simulink model "gtm_design"  (R2021b)
settings: Solver=VariableStepAuto  StartTime=0.0  StopTime=30  MinStep=0.0049  RelTol=1e-3
StopFcn:
  | MWSout=grabmws(bdroot);
  | MWSout.lastrun=datestr(now);
values from neighbouring files (symbols this model uses):
  g = 32.17405    [SingleDOF.m]    (also in layer1atm.m; mainSimple.m = 32.174; simio.m = [dx(Index.EOM(1:6)); delta(:)-f; -delta(:)-f ])
  GuidanceMode = 1    [mainSimple.m]    (also in setup.m)
  knots2fps = 1/fps2knots    (= 1.687800745)    [main.m]    (also in mainSimple.m = 1.68781)
  s = tf('s')    [SingleDOF.m]    (also in main.m; mainSimple.m; newmain.m)
undefined symbols (not defined in the file or in its folder): Aero, aftfuel, aftfuel_pos, AILL, AILLC, AILR, AILRC, alpha_deg, altitude_ft, Ax_g, Ay_g, Az_g, b, beta_deg, bias, BRAKEC, Cbar, cg_pos0, cg_shift_gear, DamageCase, DamageModels, DamageOnsetTime, Earth, ELLIB, ELLIBC, ELLOB, ELLOBC, ELRIB, ELRIBC, ELROB, ELROBC, engl_ang, engl_pos, engr_ang, engr_pos, FLAPLC, FLAPLIB, FLAPLOB, FLAPRC, FLAPRIB, FLAPROB, FuelUsed_Init, fwdfuel, fwdfuel_pos, GEAR, GEARC, Inertia0, Inertia_shift_gear, Ixx_model, Iyy_model, Izz_model, KTAS, LandingGear, LengON, LinearizeModeOn, m, MORPHLC, MORPHRC, NAV_altitude_m, NAV_latitude_deg ... (+51)
libraries: simulink_extras x39, simulink_need_slupdate x30, LPVBlockLibrary x9, aerolibconvert2 x7, simulink x3, aerolibtransform2 x3, UserContent_lib x2, uavalgslib x2, robotcorelib x1, uavutilslib x1
(part 2 of 7)

== system gtm_design/GTM_T2/Landing Gear ==
  State : Inport
  Surfaces : Inport  Port=2
  ACParams : Inport  Port=3
  Bus Selector : BusSelector  OutputSignals=BRAKE,STEER,GEAR
  Bus Selector1 : BusSelector  OutputSignals=pb,qb,rb  OutputAsBus=on
  Bus Selector2 : BusSelector  OutputSignals=ub,vb,wb  OutputAsBus=on
  Bus Selector3 : BusSelector  OutputSignals=psi
  Bus Selector4 : BusSelector  OutputSignals=altitude
  Bus Selector5 : BusSelector  OutputSignals=phi,theta,psi  OutputAsBus=on
  Bus Selector6 : BusSelector  OutputSignals=CG  OutputAsBus=on
  Bus to Vector : BusToVector
  Bus to Vector1 : BusToVector
  Bus to Vector2 : BusToVector
  Gain : Gain  Gain=1/100
  LandingGear : Subsystem  mask{NoseWheelPos=LandingGear.NoseWheelPos, LeftMainPos=LandingGear.LeftMainPos, RightMainPos=LandingGear.RightMainPos, SpringConst=LandingGear.SpringConst, DampingConst=LandingGear.DampingConst, StrokeLength=LandingGear.StrokeLength, MountStiffness=LandingGear.MountStiff, MountDamping=LandingGear.MountDamping, RunwayAlt=runway_alt}
      mask prompts: NoseWheelPos "Nose Wheel Position [X,Y,Z]"; LeftMainPos "Left Main Position [X,Y,Z]"; RightMainPos "Right Main Position [X,Y,Z]"; SpringConst "Spring Constant [Nose,Left,Right]"; DampingConst "Damping Constant [Nose,Left,Right]"; StrokeLength "Stroke Length [Nose,Left,Right]"; MountStiffness "Mount Stiffness [Nose,Left,Right]"; MountDamping "Mount Damping [Nose,Left, Right]"; RunwayAlt "Runway Altitude"
      mask help:
      | Implements ground reaction force (if geardown is nonzero) for 3-wheel landing gear. Linear stiffness and damping are applied within stroke range, and (generally larger) mount stiffness and damping are applied beyond this range.
      |
      | Underlying gear.c function is from HL-20/LaRCsim, e.b.jackson@nasa.gov
  Mux : Mux  Inputs=2
  FM : Outport
  GearState : Outport  Port=2
  wires:
  Mux/1 -> FM/1
  Gain/1 -> LandingGear/7(Brake (0-1))
  LandingGear/3(Contact) -> GearState/1
  LandingGear/2(M_gear) -> Mux/2
  LandingGear/1(F_gear) -> Mux/1
  Bus Selector/3 -> LandingGear/9(geardown (0/1))  "<GEAR>"
  Bus Selector/2 -> LandingGear/8(Steer (deg))  "<STEER>"
  Bus Selector/1 -> Gain/1  "<BRAKE>"
  Bus Selector3/1 -> LandingGear/6(Heading (Rad))  "<psi>"
  Bus to Vector/1 -> LandingGear/4(pqr (Rad/sec))
  Bus Selector4/1 -> LandingGear/3(Altitude (ft))  "<altitude>"
  Bus to Vector2/1 -> LandingGear/2(EulerAngles (Rad))
  Bus Selector6/1 -> LandingGear/1(cg)
  Surfaces/1 -> Bus Selector/1
  State/1 -> Bus Selector1/1, Bus Selector2/1, Bus Selector3/1, Bus Selector4/1, Bus Selector5/1
  Bus Selector1/1 -> Bus to Vector/1
  Bus to Vector1/1 -> LandingGear/5(Vbody (ft/sec))
  Bus Selector2/1 -> Bus to Vector1/1
  Bus Selector5/1 -> Bus to Vector2/1
  ACParams/1 -> Bus Selector6/1

== system gtm_design/GTM_T2/Sensors ==
  EOM_State : Inport
  EOM_Xdot : Inport  Port=2
  AC_Params : Inport  Port=3
  AuxVars : Inport  Port=4
  SurfacePos : Inport  Port=5
  Engines : Inport  Port=6
  Air Data : Subsystem
  AuxVars1 : InportShadow  Port=4
  Bus Creator : BusCreator  Inputs=5
  Engine ECU 8 Hz : Subsystem  SystemSampleTime=round(1/Timestep/8)*Timestep
  MAG3 IMU : Subsystem
  MIDG II 50 Hz : Subsystem  SystemSampleTime=round(1/Timestep/50)*Timestep
  Scope{,1..4} (5 alike) : Scope
  Surface Pots : Subsystem
  Terminator : Terminator
  Terminator1 : Terminator
  Sensors : Outport
  wires:
  AC_Params/1 -> Terminator1/1
  EOM_Xdot/1 -> Terminator/1
  Bus Creator/1 -> Sensors/1
  Air Data/1(AirData) -> Scope/1, Bus Creator/1  "AirData"
  MIDG II 50 Hz/1(MIDG) -> Scope1/1, Bus Creator/2  "MIDG"
  Surface Pots/1(Pots) -> Scope3/1, Bus Creator/4  "SurfacePos"
  Engine ECU 8 Hz/1(ECU) -> Scope4/1, Bus Creator/5  "Engines"
  MAG3 IMU/1(MAG3) -> Scope2/1, Bus Creator/3  "MAG3"
  Engines/1 -> Engine ECU 8 Hz/1(Engines)
  SurfacePos/1 -> Surface Pots/1(SurfacePos)
  AuxVars/1 -> Air Data/2(AuxVars), MIDG II 50 Hz/1(AuxVars)
  EOM_State/1 -> MIDG II 50 Hz/2(EOM_State), Air Data/1(EOM_State), MAG3 IMU/2(EOM_State)
  AuxVars1/1 -> MAG3 IMU/1(AuxVars)

== system gtm_design/GTM_T2/TransportDelay ==
  note: Uplink Path
  note: Downlink Path
  Sensors : Inport
  UL : Inport  Port=2
  AntiAliasing : Subsystem
  Transport Delay on Bus : Subsystem
  Transport Delay on Bus1 : Subsystem
  cmds : Outport
  DL : Outport  Port=2
  wires:
  AntiAliasing/1(O) -> Transport Delay on Bus/1(In)
  Transport Delay on Bus/1(Out) -> DL/1
  UL/1 -> Transport Delay on Bus1/1(In)
  Sensors/1 -> AntiAliasing/1(I)
  Transport Delay on Bus1/1(Out) -> cmds/1

== system gtm_design/Guidance/Airspeed Step ==
  Action Port : ActionPort  ActionPortLabel=case [ 3 ]:
  Bus Creator : BusCreator  Inputs=5
  Constant1 : Constant  Value=-12.5
  Constant2 : Constant  Value=0
  Constant3 : Constant  Value=0
  Constant4 : Constant  Value=0
  Step1 : Step  Time=5  Before=85  After=90  SampleTime=0
  GuidanceCommand : Outport  InitialOutput=zeros(5,1)
  wires:
  Constant2/1 -> Bus Creator/2  "alt_c_ft"
  Constant4/1 -> Bus Creator/4  "phi_c_deg"
  Bus Creator/1 -> GuidanceCommand/1
  Constant3/1 -> Bus Creator/3  "bet_c_deg"
  Step1/1 -> Bus Creator/1  "tas_c_knot"
  Constant1/1 -> Bus Creator/5  "etas_c_percent"

== system gtm_design/Guidance/Elevation Step ==
  Action Port : ActionPort  ActionPortLabel=case [ 2 ]:
  Bus Creator : BusCreator  Inputs=5
  Constant : Constant  Value=85
  Constant1 : Constant  Value=-12.5
  Constant3 : Constant  Value=0
  Constant4 : Constant  Value=0
  Step : Step  Time=5  After=10  SampleTime=0
  GuidanceCommand : Outport  InitialOutput=zeros(5,1)
  wires:
  Constant/1 -> Bus Creator/1  "tas_c_knot"
  Constant1/1 -> Bus Creator/5  "etas_c_percent"
  Constant3/1 -> Bus Creator/3  "bet_c_deg"
  Constant4/1 -> Bus Creator/4  "phi_c_deg"
  Bus Creator/1 -> GuidanceCommand/1
  Step/1 -> Bus Creator/2  "alt_c_ft"

== system gtm_design/Guidance/Invalid, Error Out ==
  Action Port : ActionPort  ActionPortLabel=default:
  Constant1 : Constant  Value=zeros(5,1)
  Constant2 : Constant  Value=0
  InvalidMode : Assertion  AssertionFailFcn="warndlg('Invalid settings for TrimMode and LinearizeMode.  Run setup.m to reset.','Warning!')"
  Out : Outport  InitialOutput=zeros(5,1)
  wires:
  Constant1/1 -> Out/1
  Constant2/1 -> InvalidMode/1

== system gtm_design/Guidance/Label ==
  I : Inport  PortDimensions=[5 1]
  Bus Creator : BusCreator  Inputs=5
  Demux : Demux  Outputs=5
  O : Outport
  wires:
  Demux/4 -> Bus Creator/4  "phi_c_deg"
  Demux/2 -> Bus Creator/2  "alt_c_ft"
  Demux/5 -> Bus Creator/5  "etas_c_percent"
  Demux/3 -> Bus Creator/3  "bet_c_deg"
  Demux/1 -> Bus Creator/1  "tas_c_knot"
  Bus Creator/1 -> O/1
  I/1 -> Demux/1

== system gtm_design/Guidance/Level Flight ==
  Action Port : ActionPort  ActionPortLabel=case [ 1 ]:
  Bus Creator : BusCreator  Inputs=5
  Constant : Constant  Value=85
  Constant1 : Constant  Value=-12.5
  Constant2 : Constant  Value=0
  Constant3 : Constant  Value=0
  Constant4 : Constant  Value=0
  GuidanceCommand : Outport  InitialOutput=zeros(5,1)
  wires:
  Bus Creator/1 -> GuidanceCommand/1
  Constant3/1 -> Bus Creator/3  "bet_c_deg"
  Constant/1 -> Bus Creator/1  "tas_c_knot"
  Constant1/1 -> Bus Creator/5  "etas_c_percent"
  Constant4/1 -> Bus Creator/4  "phi_c_deg"
  Constant2/1 -> Bus Creator/2  "alt_c_ft"

== system gtm_design/Guidance/Orbit Following ==
  Feedback : Inport
  Action Port : ActionPort  ActionPortLabel=case [ 6 ]:
  Bus Creator : BusCreator  Inputs=5
  Bus Selector : BusSelector  OutputSignals=North,East,Height,HeadingAngle
  Constant : Constant  Value=80
  Constant1 : Constant  Value=-12.5
  Constant2 : Constant
  Constant3 : Constant  Value=0
  Constant4 : Constant  Value=1000
  Constant5 : Constant  Value=2000
  Gain2 : Gain  Gain=-1
  Gain5 : Gain  Gain=-1
  Heading Control : MATLAB Function  TreatAsAtomicUnit=on  mask(Fixed Wing Heading Controller){PHeadingAngle=3.9}
      mask prompts: PHeadingAngle "Heading Control Gain"
      mask help: P controller that regulates fixed wing UAV heading direction through controlling its roll angle. This controller requires that the plane is flying under coordinated flight condition.
  Length Conversion : aerolibconvert2/Length Conversion  IU=m  OU=ft
  Orbit Follower : uavalgslib/Orbit Follower  UAVType=fixed-wing  MinOrbitRadius=1  MinLookaheadDistance=0.1  ExternalReset=none  ShowCrossTrackErrorOutput=off  ShowNumTurnsOutput=off  SimulateUsing=Interpreted execution
      settings: SourceProductBaseCode=UV
  Radians to Degrees : simulink_extras/Transformations/Radians to Degrees
  Saturation1 : Saturate  UpperLimit=30  LowerLimit=-30
  Selector1 : Selector  InputPortWidth=3  IndexOptions=Index vector (dialog)  Indices=[3]  OutputSizes=1
  Signal Conversion : SignalConversion  OverrideOpt=off
  Signal Conversion1 : SignalConversion  OverrideOpt=off
  Subsystem1 : Subsystem
  Terminator3 : Terminator
  Terminator4 : Terminator
  Terminator5 : Terminator
  Vector Concatenate : Concatenate  NumInputs=4
  Waypoints1 : Constant  Value=[0;3000;0]  VectorParams1D=off
  Windless : Subsystem  VariantControl=NoWind
      settings: PortSchema="{\"entries\":[{\"content\":{\"sides\":[{\"content\":{\"connectorIds\":[\"Out1\"]},\"type\":\"ConnectorPlacement.EquallySpacedRectSide\",\"uuid\":\"203a2d2a-30ae-46d5-b636-10933e29d1fa\"},{\"content\":{\"connectorIds\":[],\"side\":\"RIGHT\"},\"type\":\"ConnectorPlacement.EquallySpacedRectSide\",\"uuid\":\"332a648b-f7fb-47c3-be36-01d9c1955b3b\"},{\"content\":{\"connectorIds\":[],\"side\":\"TOP\"},\"type\":\"ConnectorPlacement.EquallySpacedRectSide\",\"uuid\":\"0294cf6c-fac0-4906-9702-b8e9ef362c1f\"}]},\"type\":\"ConnectorPlacement.EquallySpacedConnector\",\"uuid\":\"f608bdaf-466f-4a8f-9e8f-8d2734bc1053\"}],\"packageUris\":[\"http://schema.mathworks.com/mf0/Connector/R2020b\"],\"version\":\"1.0\"}"
  GuidanceCommand : Outport  InitialOutput=zeros(5,1)
  LookaheadPoint : Outport  Port=2  InitialOutput=zeros(3,1)
  DesiredCourse : Outport  Port=3  InitialOutput=zeros(1,1)
  wires:
  Radians to Degrees/1 -> Saturation1/1
  Length Conversion/1 -> Bus Creator/2  "alt_c_ft"
  Saturation1/1 -> Bus Creator/4  "phi_c_deg"
  Constant5/1 -> Orbit Follower/3
  Selector1/1 -> Gain5/1
  Constant4/1 -> Orbit Follower/5
  Subsystem1/1(Out2) -> Heading Control/1(FlightState)  "FlightState"
  Constant2/1 -> Orbit Follower/4
  Gain5/1 -> Length Conversion/1  "Height"
  Constant1/1 -> Bus Creator/5  "etas_c_percent"
  Subsystem1/2(Out1) -> Bus Selector/1
  Waypoints1/1 -> Orbit Follower/2
  Orbit Follower/4 -> Terminator4/1
  Orbit Follower/3 -> Terminator3/1
  Heading Control/1(RollAngle) -> Radians to Degrees/1  "phi_c_rad"
  Orbit Follower/1 -> Signal Conversion/1, Selector1/1
  Orbit Follower/5 -> Terminator5/1
  Gain2/1 -> Vector Concatenate/3
  Constant/1 -> Bus Creator/1  "tas_c_knot"
  Windless/1(Environment) -> Heading Control/3(e)
  Constant3/1 -> Bus Creator/3  "bet_c_deg"
  Bus Selector/3 -> Gain2/1  "<Height>"
  Bus Selector/4 -> Vector Concatenate/4  "<HeadingAngle>"
  Bus Selector/1 -> Vector Concatenate/1  "<North>"
  Orbit Follower/2 -> Signal Conversion1/1, Heading Control/2(UHeading)
  Vector Concatenate/1 -> Orbit Follower/1
  Bus Selector/2 -> Vector Concatenate/2  "<East>"
  Bus Creator/1 -> GuidanceCommand/1
  Feedback/1 -> Subsystem1/1(Feedback)
  Signal Conversion/1 -> LookaheadPoint/1
  Signal Conversion1/1 -> DesiredCourse/1

== system gtm_design/Guidance/Roll Step ==
  Action Port : ActionPort  ActionPortLabel=case [ 4 ]:
  Bus Creator : BusCreator  Inputs=5
  Constant1 : Constant  Value=-12.5
  Constant2 : Constant  Value=0
  Constant4 : Constant  Value=0
  Constant5 : Constant  Value=85
  Step2 : Step  Time=5  After=20  SampleTime=0
  GuidanceCommand : Outport  InitialOutput=zeros(5,1)
  wires:
  Constant1/1 -> Bus Creator/5  "etas_c_percent"
  Constant4/1 -> Bus Creator/3  "bet_c_deg"
  Constant2/1 -> Bus Creator/2  "alt_c_ft"
  Step2/1 -> Bus Creator/4  "phi_c_deg"
  Bus Creator/1 -> GuidanceCommand/1
  Constant5/1 -> Bus Creator/1  "tas_c_knot"

== system gtm_design/Guidance/Waypoint Following ==
  Feedback : Inport
  Action Port : ActionPort  ActionPortLabel=case [ 5 ]:
  Bus Creator : BusCreator  Inputs=5
  Bus Selector : BusSelector  OutputSignals=North,East,Height,HeadingAngle
  Constant : Constant  Value=80
  Constant1 : Constant  Value=-12.5
  Constant3 : Constant  Value=0
  Constant4 : Constant  Value=1000
  Gain2 : Gain  Gain=-1
  Gain5 : Gain  Gain=-1
  Heading Control : MATLAB Function  TreatAsAtomicUnit=on  mask(Fixed Wing Heading Controller){PHeadingAngle=3.9}
      mask prompts: PHeadingAngle "Heading Control Gain"
      mask help: P controller that regulates fixed wing UAV heading direction through controlling its roll angle. This controller requires that the plane is flying under coordinated flight condition.
  Length Conversion : aerolibconvert2/Length Conversion  IU=m  OU=ft
  Radians to Degrees : simulink_extras/Transformations/Radians to Degrees
  Saturation1 : Saturate  UpperLimit=30  LowerLimit=-30
  Selector1 : Selector  InputPortWidth=3  IndexOptions=Index vector (dialog)  Indices=[3]  OutputSizes=1
  Signal Conversion : SignalConversion  OverrideOpt=off
  Signal Conversion1 : SignalConversion  OverrideOpt=off
  Subsystem1 : Subsystem
  Terminator3 : Terminator
  Terminator4 : Terminator
  Vector Concatenate : Concatenate  NumInputs=4
  Waypoint Follower : uavalgslib/Waypoint Follower  UAVType=fixed-wing  StartFrom=first  TransitionRadiusSource=internal  TransitionRadius=100  MinLookaheadDistance=0.1  YawInput=off  ShowCrossTrackErrorOutput=off  ShowStatusOutput=off  SimulateUsing=Interpreted execution
      settings: SourceProductBaseCode=UV
  Waypoints : Constant  Value=[0;3000;0]  VectorParams1D=off
  Windless : Subsystem  VariantControl=NoWind
      settings: PortSchema="{\"entries\":[{\"content\":{\"sides\":[{\"content\":{\"connectorIds\":[\"Out1\"]},\"type\":\"ConnectorPlacement.EquallySpacedRectSide\",\"uuid\":\"203a2d2a-30ae-46d5-b636-10933e29d1fa\"},{\"content\":{\"connectorIds\":[],\"side\":\"RIGHT\"},\"type\":\"ConnectorPlacement.EquallySpacedRectSide\",\"uuid\":\"332a648b-f7fb-47c3-be36-01d9c1955b3b\"},{\"content\":{\"connectorIds\":[],\"side\":\"TOP\"},\"type\":\"ConnectorPlacement.EquallySpacedRectSide\",\"uuid\":\"0294cf6c-fac0-4906-9702-b8e9ef362c1f\"}]},\"type\":\"ConnectorPlacement.EquallySpacedConnector\",\"uuid\":\"f608bdaf-466f-4a8f-9e8f-8d2734bc1053\"}],\"packageUris\":[\"http://schema.mathworks.com/mf0/Connector/R2020b\"],\"version\":\"1.0\"}"
  GuidanceCommand : Outport  InitialOutput=zeros(5,1)
  LookaheadPoint : Outport  Port=2  InitialOutput=zeros(3,1)
  DesiredCourse : Outport  Port=3  InitialOutput=zeros(1,1)
  wires:
  Feedback/1 -> Subsystem1/1(Feedback)
  Bus Creator/1 -> GuidanceCommand/1
  Bus Selector/2 -> Vector Concatenate/2  "<East>"
  Vector Concatenate/1 -> Waypoint Follower/1
  Waypoint Follower/2 -> Signal Conversion1/1, Heading Control/2(UHeading)
  Bus Selector/1 -> Vector Concatenate/1  "<North>"
  Bus Selector/4 -> Vector Concatenate/4  "<HeadingAngle>"
  Bus Selector/3 -> Gain2/1  "<Height>"
  Constant3/1 -> Bus Creator/3  "bet_c_deg"
  Windless/1(Environment) -> Heading Control/3(e)
  Constant/1 -> Bus Creator/1  "tas_c_knot"
  Gain2/1 -> Vector Concatenate/3
  Waypoint Follower/1 -> Selector1/1, Signal Conversion/1
  Heading Control/1(RollAngle) -> Radians to Degrees/1  "phi_c_rad"
  Waypoint Follower/3 -> Terminator3/1
  Waypoint Follower/4 -> Terminator4/1
  Waypoints/1 -> Waypoint Follower/2
  Subsystem1/2(Out1) -> Bus Selector/1
  Constant1/1 -> Bus Creator/5  "etas_c_percent"
  Gain5/1 -> Length Conversion/1  "Height"
  Subsystem1/1(Out2) -> Heading Control/1(FlightState)  "FlightState"
  Constant4/1 -> Waypoint Follower/3
  Selector1/1 -> Gain5/1
  Saturation1/1 -> Bus Creator/4  "phi_c_deg"
  Length Conversion/1 -> Bus Creator/2  "alt_c_ft"
  Radians to Degrees/1 -> Saturation1/1
  Signal Conversion/1 -> LookaheadPoint/1
  Signal Conversion1/1 -> DesiredCourse/1

== system gtm_design/Control/BiasSurfs/Label ==
  In1 : Inport
  Bus Creator : BusCreator  Inputs=21
  Demux : Demux  Outputs=21
  UL : Outport
  wires:
  Demux/21 -> Bus Creator/21  "STEERC"
  Demux/19 -> Bus Creator/19  "GEARC"
  Demux/18 -> Bus Creator/18  "MORPHRC"
  Demux/2 -> Bus Creator/2  "THROTRC"
  Demux/6 -> Bus Creator/6  "ELRIBC"
  Demux/14 -> Bus Creator/14  "SPLROBC"
  Demux/7 -> Bus Creator/7  "AILLC"
  Demux/15 -> Bus Creator/15  "FLAPLC"
  Demux/10 -> Bus Creator/10  "RUDLOC"
  Demux/16 -> Bus Creator/16  "MORPHLC"
  Demux/12 -> Bus Creator/12  "SPLLOBC"
  Demux/9 -> Bus Creator/9  "RUDUPC"
  Bus Creator/1 -> UL/1
  Demux/11 -> Bus Creator/11  "SPLLIBC"
  In1/1 -> Demux/1
  Demux/13 -> Bus Creator/13  "SPLRIBC"
  Demux/1 -> Bus Creator/1  "THROTLC"
  Demux/5 -> Bus Creator/5  "ELROBC"
  Demux/8 -> Bus Creator/8  "AILRC"
  Demux/4 -> Bus Creator/4  "ELLIBC"
  Demux/20 -> Bus Creator/20  "BRAKEC"
  Demux/17 -> Bus Creator/17  "FLAPRC"
  Demux/3 -> Bus Creator/3  "ELLOBC"

== system gtm_design/Control/Controller/Bias Mixer ==
  In : Inport
  Display : Display
  Elevator : Constant  Value=bias.elevator
  Flaps1 : Constant  Value=bias.rudder
  Flaps2 : Constant  Value=bias.aileron
  Flaps3 : Constant  Value=bias.morphing
  Flaps4 : Constant  Value=bias.morphing
  Mux : Mux  Inputs=6
  Sum : Sum  Inputs=|+-
  Throttle : Constant  Value=bias.throttle
  Out : Outport
  wires:
  Throttle/1 -> Mux/1
  Elevator/1 -> Mux/2
  Flaps2/1 -> Mux/3
  Flaps1/1 -> Mux/4
  Flaps3/1 -> Mux/5
  Flaps4/1 -> Mux/6
  In/1 -> Sum/1
  Mux/1 -> Sum/2, Display/1
  Sum/1 -> Out/1

== system gtm_design/Control/Controller/Control Algorithm ==
  cmd_guid : Inport
  feedback : Inport  Port=2
  Lateral-Directional Controller : Subsystem
  Longitudinal Controller : Subsystem
  Longitudinal Controller (Gamma) : Subsystem  Commented=on
  cmd_guid1 : InportShadow
  feedback1 : InportShadow  Port=2
  THROTC : Outport
  ELLC : Outport  Port=2
  AILC : Outport  Port=3
  RUDC : Outport  Port=4
  SPANAC : Outport  Port=5
  wires:
  feedback/1 -> Longitudinal Controller/2(feedback)
  cmd_guid/1 -> Longitudinal Controller/1(cmd_guid)
  Longitudinal Controller/2(ELLC) -> ELLC/1  "dele_c_deg"
  Longitudinal Controller/1(THROTC) -> THROTC/1  "delt_c_percent"
  Lateral-Directional Controller/1(AILC) -> AILC/1
  Lateral-Directional Controller/2(RUDC) -> RUDC/1
  cmd_guid1/1 -> Lateral-Directional Controller/1(cmd_guid)
  feedback1/1 -> Lateral-Directional Controller/2(feedback)
  Lateral-Directional Controller/3(SPANAC) -> SPANAC/1

== system gtm_design/Control/Controller/Morphing Mixer ==
  SPANAC : Inport
  SPANSC : Inport  Port=2
  Add : Sum
  Subtract : Sum  Inputs=+-
  SPANLC : Outport
  SPANRC : Outport  Port=2
  wires:
  SPANSC/1 -> Subtract/1, Add/2
  SPANAC/1 -> Add/1, Subtract/2
  Subtract/1 -> SPANLC/1
  Add/1 -> SPANRC/1

== system gtm_design/GTM_T2/A//C parameters/Inertia//Mass//CG Shift ==
  note: Inertia "vector" = [Ixx Iyy Izz Ixz Iyz Ixy]
  gear : Inport
  fuel_used : Inport  Port=2
  DamageCase : Inport  Port=3
  morphing : Inport  Port=4
  Add : Sum
  Add1 : Sum  Inputs=+++++
  Add2 : Sum  Inputs=++++
  Add3 : Sum  Inputs=-+
  DamageEffects : Subsystem
  Divide1 : Product  Inputs=/*
  FuelBurnEffects : Subsystem
  Gain : Gain  Gain=1/32.17405
  MorphingEffects : Subsystem  Commented=on
  MorphingEffects1 : Subsystem  Commented=on
  Reshape : Reshape
  Reshape1 : Reshape
  Switch : Switch  Threshold=0.5
  Switch1 : Switch  Threshold=0.5
  cg/weight : Subsystem
  "fuel cg shift, cg_pos0" : MATLAB Function  TreatAsAtomicUnit=on
  ixxb3 : Constant  Value=Inertia0
  ixxb7 : Constant  Value=w0
  xCG1 : Constant  Value=zeros(1,3)
  xCG3 : Constant  Value=Inertia_shift_gear
  xCG4 : Constant  Value=cg_shift_gear
  xCG5 : Constant  Value=zeros(1,6)
  Inertia : Outport
  mass : Outport  Port=2
  CG : Outport  Port=3
  wires:
  "fuel cg shift, cg_pos0"/1(y) -> Divide1/2
  Divide1/1 -> Add2/2
  Reshape1/1 -> Inertia/1
  Reshape/1 -> CG/1
  cg/weight/2(dweight) -> Add/1
  gear/1 -> Switch1/2, Switch/2
  cg/weight/1(dCG) -> Add2/1
  Add3/1 -> Add/2
  xCG1/1 -> Switch1/3
  xCG4/1 -> Switch1/1
  Switch1/1 -> Add2/3
  ixxb7/1 -> Add3/2
  Gain/1 -> mass/1
  Add2/1 -> Reshape/1
  Add/1 -> Divide1/1, Gain/1  "gwest"
  DamageCase/1 -> cg/weight/1(DamageCase), DamageEffects/1(In)
  DamageEffects/1(dInertia) -> Add1/3
  ixxb3/1 -> Add1/4
  fuel_used/1 -> "fuel cg shift, cg_pos0"/1(fuel_used), Add3/1, FuelBurnEffects/1(In)
  xCG5/1 -> Switch/3
  xCG3/1 -> Switch/1
  Add1/1 -> Reshape1/1
  Switch/1 -> Add1/1
  FuelBurnEffects/1(dInertia) -> Add1/2
  morphing/1 -> MorphingEffects1/1(morphing), MorphingEffects/1(morphing)
  MorphingEffects/1(dInertia) -> Add1/5
  MorphingEffects1/1(dCG) -> Add2/4

== system gtm_design/GTM_T2/A//C parameters/TriggerDamage ==
  Clock : Clock
  DamgeCase : Constant  Value=DamageCase
  Switch : Switch  Threshold=DamageOnsetTime
  Zero : Constant  Value=0
  damagecase : Outport
  wires:
  Clock/1 -> Switch/2
  Switch/1 -> damagecase/1
  Zero/1 -> Switch/3
  DamgeCase/1 -> Switch/1

== system gtm_design/GTM_T2/Actuators/Acutator Dynamics ==
  In : Inport
  Brake : Saturate  UpperLimit=100  LowerLimit=0
  Bus Selector2 : BusSelector  OutputSignals=ELLOBC,ELLIBC,ELROBC,ELRIBC,AILLC,AILRC,RUDUPC,RUDLOC,SPLLIBC,SPLLOBC,SPLRIBC,SPLROBC,FLAPLC,MORPHLC,FLAPRC,MORPHRC,GEARC,BRAKEC,THROTLC,THROTRC,STEERC
  ElevatorLIBServo : Subsystem  mask(Rate and Position Limited Servo){freq=5, RL=300, POS_hi=20, POS_lo=-30, Bias=bias.elevator}
      mask prompts: freq "Bandwidth, Hz"; RL "Rate Limit:"; POS_hi "Position Limit High:"; POS_lo "Position Limit Low:"; Bias "Bias Value:"
      mask help:
      | First order transfer function: w/(s+w), with rate and position limits
      | and output bias level.
      mask Display:
      | text(.48,.55,sprintf('%3.1f Hz\nBW',freq),'horizontalAlignment','center');
      | 
      | text(0.18,0.45,sprintf('|d/dt|\n<%0.1f',RL),'horizontalAlignment','center');
      | 
      | text(0.88,0.85,num2str(POS_hi),'horizontalAlignment', 'center');
      | text(0.88,0.2,num2str(POS_lo),'horizontalAlignment', 'center');
      | text(0.73,0.5,'P\nL');
      | 
      | 
      | plot([0.83 0.87 0.93 0.97],[0.4 0.4 0.6 0.6]);
      | plot([0.81 0.99],[0.5 0.5]);
      | plot([0.9 0.9],[0.3 0.7]);
      | plot([0.81 0.99 0.99 0.81 0.81],[0.3 0.3 0.7 0.7 0.3]);
  ElevatorLOBServo : Subsystem  mask(Rate and Position Limited Servo){freq=5, RL=300, POS_hi=20, POS_lo=-30, Bias=bias.elevator}
      mask prompts: freq "Bandwidth, Hz"; RL "Rate Limit:"; POS_hi "Position Limit High:"; POS_lo "Position Limit Low:"; Bias "Bias Value:"
      mask help:
      | First order transfer function: w/(s+w), with rate and position limits
      | and output bias level.
      mask Display:
      | text(.48,.55,sprintf('%3.1f Hz\nBW',freq),'horizontalAlignment','center');
      | 
      | text(0.18,0.45,sprintf('|d/dt|\n<%0.1f',RL),'horizontalAlignment','center');
      | 
      | text(0.88,0.85,num2str(POS_hi),'horizontalAlignment', 'center');
      | text(0.88,0.2,num2str(POS_lo),'horizontalAlignment', 'center');
      | text(0.73,0.5,'P\nL');
      | 
      | 
      | plot([0.83 0.87 0.93 0.97],[0.4 0.4 0.6 0.6]);
      | plot([0.81 0.99],[0.5 0.5]);
      | plot([0.9 0.9],[0.3 0.7]);
      | plot([0.81 0.99 0.99 0.81 0.81],[0.3 0.3 0.7 0.7 0.3]);
  ElevatorRIBServo : Subsystem  mask(Rate and Position Limited Servo){freq=5, RL=300, POS_hi=20, POS_lo=-30, Bias=bias.elevator}
      mask prompts: freq "Bandwidth, Hz"; RL "Rate Limit:"; POS_hi "Position Limit High:"; POS_lo "Position Limit Low:"; Bias "Bias Value:"
      mask help:
      | First order transfer function: w/(s+w), with rate and position limits
      | and output bias level.
      mask Display:
      | text(.48,.55,sprintf('%3.1f Hz\nBW',freq),'horizontalAlignment','center');
      | 
      | text(0.18,0.45,sprintf('|d/dt|\n<%0.1f',RL),'horizontalAlignment','center');
      | 
      | text(0.88,0.85,num2str(POS_hi),'horizontalAlignment', 'center');
      | text(0.88,0.2,num2str(POS_lo),'horizontalAlignment', 'center');
      | text(0.73,0.5,'P\nL');
      | 
      | 
      | plot([0.83 0.87 0.93 0.97],[0.4 0.4 0.6 0.6]);
      | plot([0.81 0.99],[0.5 0.5]);
      | plot([0.9 0.9],[0.3 0.7]);
      | plot([0.81 0.99 0.99 0.81 0.81],[0.3 0.3 0.7 0.7 0.3]);
  ElevatorROBServo : Subsystem  mask(Rate and Position Limited Servo){freq=5, RL=300, POS_hi=20, POS_lo=-30, Bias=bias.elevator}
      mask prompts: freq "Bandwidth, Hz"; RL "Rate Limit:"; POS_hi "Position Limit High:"; POS_lo "Position Limit Low:"; Bias "Bias Value:"
      mask help:
      | First order transfer function: w/(s+w), with rate and position limits
      | and output bias level.
      mask Display:
      | text(.48,.55,sprintf('%3.1f Hz\nBW',freq),'horizontalAlignment','center');
      | 
      | text(0.18,0.45,sprintf('|d/dt|\n<%0.1f',RL),'horizontalAlignment','center');
      | 
      | text(0.88,0.85,num2str(POS_hi),'horizontalAlignment', 'center');
      | text(0.88,0.2,num2str(POS_lo),'horizontalAlignment', 'center');
      | text(0.73,0.5,'P\nL');
      | 
      | 
      | plot([0.83 0.87 0.93 0.97],[0.4 0.4 0.6 0.6]);
      | plot([0.81 0.99],[0.5 0.5]);
      | plot([0.9 0.9],[0.3 0.7]);
      | plot([0.81 0.99 0.99 0.81 0.81],[0.3 0.3 0.7 0.7 0.3]);
  FlapLServo : Subsystem  mask(Rate and Position Limited Servo){freq=5, RL=300, POS_hi=30, POS_lo=0, Bias=bias.morphing}
      mask prompts: freq "Bandwidth, Hz"; RL "Rate Limit:"; POS_hi "Position Limit High:"; POS_lo "Position Limit Low:"; Bias "Bias Value:"
      mask help:
      | First order transfer function: w/(s+w), with rate and position limits
      | and output bias level.
      mask Display:
      | text(.48,.55,sprintf('%3.1f Hz\nBW',freq),'horizontalAlignment','center');
      | 
      | text(0.18,0.45,sprintf('|d/dt|\n<%0.1f',RL),'horizontalAlignment','center');
      | 
      | text(0.88,0.85,num2str(POS_hi),'horizontalAlignment', 'center');
      | text(0.88,0.2,num2str(POS_lo),'horizontalAlignment', 'center');
      | text(0.73,0.5,'P\nL');
      | 
      | 
      | plot([0.83 0.87 0.93 0.97],[0.4 0.4 0.6 0.6]);
      | plot([0.81 0.99],[0.5 0.5]);
      | plot([0.9 0.9],[0.3 0.7]);
      | plot([0.81 0.99 0.99 0.81 0.81],[0.3 0.3 0.7 0.7 0.3]);
  FlapRServo : Subsystem  mask(Rate and Position Limited Servo){freq=5, RL=300, POS_hi=30, POS_lo=0, Bias=bias.morphing}
      mask prompts: freq "Bandwidth, Hz"; RL "Rate Limit:"; POS_hi "Position Limit High:"; POS_lo "Position Limit Low:"; Bias "Bias Value:"
      mask help:
      | First order transfer function: w/(s+w), with rate and position limits
      | and output bias level.
      mask Display:
      | text(.48,.55,sprintf('%3.1f Hz\nBW',freq),'horizontalAlignment','center');
      | 
      | text(0.18,0.45,sprintf('|d/dt|\n<%0.1f',RL),'horizontalAlignment','center');
      | 
      | text(0.88,0.85,num2str(POS_hi),'horizontalAlignment', 'center');
      | text(0.88,0.2,num2str(POS_lo),'horizontalAlignment', 'center');
      | text(0.73,0.5,'P\nL');
      | 
      | 
      | plot([0.83 0.87 0.93 0.97],[0.4 0.4 0.6 0.6]);
      | plot([0.81 0.99],[0.5 0.5]);
      | plot([0.9 0.9],[0.3 0.7]);
      | plot([0.81 0.99 0.99 0.81 0.81],[0.3 0.3 0.7 0.7 0.3]);
  Gear : Saturate  UpperLimit=1  LowerLimit=0
  L Throttle : Saturate  UpperLimit=100  LowerLimit=0
  LeftAileronServo : Subsystem  mask(Rate and Position Limited Servo){freq=5, RL=300, POS_hi=20.0, POS_lo=-20, Bias=-1*bias.aileron}
      mask prompts: freq "Bandwidth, Hz"; RL "Rate Limit:"; POS_hi "Position Limit High:"; POS_lo "Position Limit Low:"; Bias "Bias Value:"
      mask help:
      | First order transfer function: w/(s+w), with rate and position limits
      | and output bias level.
      mask Display:
      | text(.48,.55,sprintf('%3.1f Hz\nBW',freq),'horizontalAlignment','center');
      | 
      | text(0.18,0.45,sprintf('|d/dt|\n<%0.1f',RL),'horizontalAlignment','center');
      | 
      | text(0.88,0.85,num2str(POS_hi),'horizontalAlignment', 'center');
      | text(0.88,0.2,num2str(POS_lo),'horizontalAlignment', 'center');
      | text(0.73,0.5,'P\nL');
      | 
      | 
      | plot([0.83 0.87 0.93 0.97],[0.4 0.4 0.6 0.6]);
      | plot([0.81 0.99],[0.5 0.5]);
      | plot([0.9 0.9],[0.3 0.7]);
      | plot([0.81 0.99 0.99 0.81 0.81],[0.3 0.3 0.7 0.7 0.3]);
  LeftIBSpoilerServo : Subsystem  mask(Rate and Position Limited Servo){freq=5, RL=300, POS_hi=15, POS_lo=0, Bias=bias.morphing}
      mask prompts: freq "Bandwidth, Hz"; RL "Rate Limit:"; POS_hi "Position Limit High:"; POS_lo "Position Limit Low:"; Bias "Bias Value:"
      mask help:
      | First order transfer function: w/(s+w), with rate and position limits
      | and output bias level.
      mask Display:
      | text(.48,.55,sprintf('%3.1f Hz\nBW',freq),'horizontalAlignment','center');
      | 
      | text(0.18,0.45,sprintf('|d/dt|\n<%0.1f',RL),'horizontalAlignment','center');
      | 
      | text(0.88,0.85,num2str(POS_hi),'horizontalAlignment', 'center');
      | text(0.88,0.2,num2str(POS_lo),'horizontalAlignment', 'center');
      | text(0.73,0.5,'P\nL');
      | 
      | 
      | plot([0.83 0.87 0.93 0.97],[0.4 0.4 0.6 0.6]);
      | plot([0.81 0.99],[0.5 0.5]);
      | plot([0.9 0.9],[0.3 0.7]);
      | plot([0.81 0.99 0.99 0.81 0.81],[0.3 0.3 0.7 0.7 0.3]);
  LeftOBSpoilerServo : Subsystem  mask(Rate and Position Limited Servo){freq=5, RL=300, POS_hi=45, POS_lo=0, Bias=bias.speedbrake}
      mask prompts: freq "Bandwidth, Hz"; RL "Rate Limit:"; POS_hi "Position Limit High:"; POS_lo "Position Limit Low:"; Bias "Bias Value:"
      mask help:
      | First order transfer function: w/(s+w), with rate and position limits
      | and output bias level.
      mask Display:
      | text(.48,.55,sprintf('%3.1f Hz\nBW',freq),'horizontalAlignment','center');
      | 
      | text(0.18,0.45,sprintf('|d/dt|\n<%0.1f',RL),'horizontalAlignment','center');
      | 
      | text(0.88,0.85,num2str(POS_hi),'horizontalAlignment', 'center');
      | text(0.88,0.2,num2str(POS_lo),'horizontalAlignment', 'center');
      | text(0.73,0.5,'P\nL');
      | 
      | 
      | plot([0.83 0.87 0.93 0.97],[0.4 0.4 0.6 0.6]);
      | plot([0.81 0.99],[0.5 0.5]);
      | plot([0.9 0.9],[0.3 0.7]);
      | plot([0.81 0.99 0.99 0.81 0.81],[0.3 0.3 0.7 0.7 0.3]);
  LeftSpanServo : Subsystem  mask(Rate and Position Limited Servo){freq=5, RL=30, POS_hi=0, POS_lo=-25, Bias=bias.morphing}
      mask prompts: freq "Bandwidth, Hz"; RL "Rate Limit:"; POS_hi "Position Limit High:"; POS_lo "Position Limit Low:"; Bias "Bias Value:"
      mask help:
      | First order transfer function: w/(s+w), with rate and position limits
      | and output bias level.
      mask Display:
      | text(.48,.55,sprintf('%3.1f Hz\nBW',freq),'horizontalAlignment','center');
      | 
      | text(0.18,0.45,sprintf('|d/dt|\n<%0.1f',RL),'horizontalAlignment','center');
      | 
      | text(0.88,0.85,num2str(POS_hi),'horizontalAlignment', 'center');
      | text(0.88,0.2,num2str(POS_lo),'horizontalAlignment', 'center');
      | text(0.73,0.5,'P\nL');
      | 
      | 
      | plot([0.83 0.87 0.93 0.97],[0.4 0.4 0.6 0.6]);
      | plot([0.81 0.99],[0.5 0.5]);
      | plot([0.9 0.9],[0.3 0.7]);
      | plot([0.81 0.99 0.99 0.81 0.81],[0.3 0.3 0.7 0.7 0.3]);
  Mux : Mux  Inputs=21
  R Throttle : Saturate  UpperLimit=100  LowerLimit=0
  RightAileronServo : Subsystem  mask(Rate and Position Limited Servo){freq=5, RL=300, POS_hi=20.0, POS_lo=-20, Bias=bias.aileron}
      mask prompts: freq "Bandwidth, Hz"; RL "Rate Limit:"; POS_hi "Position Limit High:"; POS_lo "Position Limit Low:"; Bias "Bias Value:"
      mask help:
      | First order transfer function: w/(s+w), with rate and position limits
      | and output bias level.
      mask Display:
      | text(.48,.55,sprintf('%3.1f Hz\nBW',freq),'horizontalAlignment','center');
      | 
      | text(0.18,0.45,sprintf('|d/dt|\n<%0.1f',RL),'horizontalAlignment','center');
      | 
      | text(0.88,0.85,num2str(POS_hi),'horizontalAlignment', 'center');
      | text(0.88,0.2,num2str(POS_lo),'horizontalAlignment', 'center');
      | text(0.73,0.5,'P\nL');
      | 
      | 
      | plot([0.83 0.87 0.93 0.97],[0.4 0.4 0.6 0.6]);
      | plot([0.81 0.99],[0.5 0.5]);
      | plot([0.9 0.9],[0.3 0.7]);
      | plot([0.81 0.99 0.99 0.81 0.81],[0.3 0.3 0.7 0.7 0.3]);
  RightIBSpoilerServo : Subsystem  mask(Rate and Position Limited Servo){freq=5, RL=300, POS_hi=15, POS_lo=0, Bias=bias.morphing}
      mask prompts: freq "Bandwidth, Hz"; RL "Rate Limit:"; POS_hi "Position Limit High:"; POS_lo "Position Limit Low:"; Bias "Bias Value:"
      mask help:
      | First order transfer function: w/(s+w), with rate and position limits
      | and output bias level.
      mask Display:
      | text(.48,.55,sprintf('%3.1f Hz\nBW',freq),'horizontalAlignment','center');
      | 
      | text(0.18,0.45,sprintf('|d/dt|\n<%0.1f',RL),'horizontalAlignment','center');
      | 
      | text(0.88,0.85,num2str(POS_hi),'horizontalAlignment', 'center');
      | text(0.88,0.2,num2str(POS_lo),'horizontalAlignment', 'center');
      | text(0.73,0.5,'P\nL');
      | 
      | 
      | plot([0.83 0.87 0.93 0.97],[0.4 0.4 0.6 0.6]);
      | plot([0.81 0.99],[0.5 0.5]);
      | plot([0.9 0.9],[0.3 0.7]);
      | plot([0.81 0.99 0.99 0.81 0.81],[0.3 0.3 0.7 0.7 0.3]);
  RightOBSpoilerServo : Subsystem  mask(Rate and Position Limited Servo){freq=5, RL=300, POS_hi=45, POS_lo=0, Bias=bias.speedbrake}
      mask prompts: freq "Bandwidth, Hz"; RL "Rate Limit:"; POS_hi "Position Limit High:"; POS_lo "Position Limit Low:"; Bias "Bias Value:"
      mask help:
      | First order transfer function: w/(s+w), with rate and position limits
      | and output bias level.
      mask Display:
      | text(.48,.55,sprintf('%3.1f Hz\nBW',freq),'horizontalAlignment','center');
      | 
      | text(0.18,0.45,sprintf('|d/dt|\n<%0.1f',RL),'horizontalAlignment','center');
      | 
      | text(0.88,0.85,num2str(POS_hi),'horizontalAlignment', 'center');
      | text(0.88,0.2,num2str(POS_lo),'horizontalAlignment', 'center');
      | text(0.73,0.5,'P\nL');
      | 
      | 
      | plot([0.83 0.87 0.93 0.97],[0.4 0.4 0.6 0.6]);
      | plot([0.81 0.99],[0.5 0.5]);
      | plot([0.9 0.9],[0.3 0.7]);
      | plot([0.81 0.99 0.99 0.81 0.81],[0.3 0.3 0.7 0.7 0.3]);
  RightSpanServo : Subsystem  mask(Rate and Position Limited Servo){freq=5, RL=30, POS_hi=0, POS_lo=-25, Bias=bias.morphing}
      mask prompts: freq "Bandwidth, Hz"; RL "Rate Limit:"; POS_hi "Position Limit High:"; POS_lo "Position Limit Low:"; Bias "Bias Value:"
      mask help:
      | First order transfer function: w/(s+w), with rate and position limits
      | and output bias level.
      mask Display:
      | text(.48,.55,sprintf('%3.1f Hz\nBW',freq),'horizontalAlignment','center');
      | 
      | text(0.18,0.45,sprintf('|d/dt|\n<%0.1f',RL),'horizontalAlignment','center');
      | 
      | text(0.88,0.85,num2str(POS_hi),'horizontalAlignment', 'center');
      | text(0.88,0.2,num2str(POS_lo),'horizontalAlignment', 'center');
      | text(0.73,0.5,'P\nL');
      | 
      | 
      | plot([0.83 0.87 0.93 0.97],[0.4 0.4 0.6 0.6]);
      | plot([0.81 0.99],[0.5 0.5]);
      | plot([0.9 0.9],[0.3 0.7]);
      | plot([0.81 0.99 0.99 0.81 0.81],[0.3 0.3 0.7 0.7 0.3]);
  RudderLServo : Subsystem  mask(Rate and Position Limited Servo){freq=5, RL=300, POS_hi=30, POS_lo=-30.0, Bias=bias.rudder}
      mask prompts: freq "Bandwidth, Hz"; RL "Rate Limit:"; POS_hi "Position Limit High:"; POS_lo "Position Limit Low:"; Bias "Bias Value:"
      mask help:
      | First order transfer function: w/(s+w), with rate and position limits
      | and output bias level.
      mask Display:
      | text(.48,.55,sprintf('%3.1f Hz\nBW',freq),'horizontalAlignment','center');
      | 
      | text(0.18,0.45,sprintf('|d/dt|\n<%0.1f',RL),'horizontalAlignment','center');
      | 
      | text(0.88,0.85,num2str(POS_hi),'horizontalAlignment', 'center');
      | text(0.88,0.2,num2str(POS_lo),'horizontalAlignment', 'center');
      | text(0.73,0.5,'P\nL');
      | 
      | 
      | plot([0.83 0.87 0.93 0.97],[0.4 0.4 0.6 0.6]);
      | plot([0.81 0.99],[0.5 0.5]);
      | plot([0.9 0.9],[0.3 0.7]);
      | plot([0.81 0.99 0.99 0.81 0.81],[0.3 0.3 0.7 0.7 0.3]);
  RudderUServo : Subsystem  mask(Rate and Position Limited Servo){freq=5, RL=300, POS_hi=30, POS_lo=-30.0, Bias=bias.rudder}
      mask prompts: freq "Bandwidth, Hz"; RL "Rate Limit:"; POS_hi "Position Limit High:"; POS_lo "Position Limit Low:"; Bias "Bias Value:"
      mask help:
      | First order transfer function: w/(s+w), with rate and position limits
      | and output bias level.
      mask Display:
      | text(.48,.55,sprintf('%3.1f Hz\nBW',freq),'horizontalAlignment','center');
      | 
      | text(0.18,0.45,sprintf('|d/dt|\n<%0.1f',RL),'horizontalAlignment','center');
      | 
      | text(0.88,0.85,num2str(POS_hi),'horizontalAlignment', 'center');
      | text(0.88,0.2,num2str(POS_lo),'horizontalAlignment', 'center');
      | text(0.73,0.5,'P\nL');
      | 
      | 
      | plot([0.83 0.87 0.93 0.97],[0.4 0.4 0.6 0.6]);
      | plot([0.81 0.99],[0.5 0.5]);
      | plot([0.9 0.9],[0.3 0.7]);
      | plot([0.81 0.99 0.99 0.81 0.81],[0.3 0.3 0.7 0.7 0.3]);
  SteeringServo : Subsystem  mask(Rate and Position Limited Servo){freq=10, RL=300, POS_hi=30, POS_lo=-30, Bias=0}
      mask prompts: freq "Bandwidth, Hz"; RL "Rate Limit:"; POS_hi "Position Limit High:"; POS_lo "Position Limit Low:"; Bias "Bias Value:"
      mask help:
      | First order transfer function: w/(s+w), with rate and position limits
      | and output bias level.
      mask Display:
      | text(.48,.55,sprintf('%3.1f Hz\nBW',freq),'horizontalAlignment','center');
      | 
      | text(0.18,0.45,sprintf('|d/dt|\n<%0.1f',RL),'horizontalAlignment','center');
      | 
      | text(0.88,0.85,num2str(POS_hi),'horizontalAlignment', 'center');
      | text(0.88,0.2,num2str(POS_lo),'horizontalAlignment', 'center');
      | text(0.73,0.5,'P\nL');
      | 
      | 
      | plot([0.83 0.87 0.93 0.97],[0.4 0.4 0.6 0.6]);
      | plot([0.81 0.99],[0.5 0.5]);
      | plot([0.9 0.9],[0.3 0.7]);
      | plot([0.81 0.99 0.99 0.81 0.81],[0.3 0.3 0.7 0.7 0.3]);
  Sum : Sum  Inputs=++|
  Sum1 : Sum  Inputs=++|
  Sum2 : Sum  Inputs=++|
  Throttle : Constant  Value=bias.throttle
  Throttle1 : Constant  Value=bias.throttle
  Throttle2 : Constant  Value=bias.geardown
  To Workspace : ToWorkspace  VariableName=control_c  SampleTime=-1
  To Workspace1 : ToWorkspace  VariableName=control  SampleTime=-1
  Out : Outport
  wires:
  Bus Selector2/17 -> Sum2/2  "<GEARC>"
  Throttle2/1 -> Sum2/1
  Sum2/1 -> Gear/1
  Bus Selector2/20 -> Sum1/2  "<THROTRC>"
  Throttle1/1 -> Sum1/1
  Sum1/1 -> R Throttle/1
  Bus Selector2/19 -> Sum/2  "<THROTLC>"
  Throttle/1 -> Sum/1
  Sum/1 -> L Throttle/1
  SteeringServo/1(Out) -> Mux/21
  R Throttle/1 -> Mux/20
  L Throttle/1 -> Mux/19
  Brake/1 -> Mux/18
  Gear/1 -> Mux/17
  Mux/1 -> To Workspace1/1, Out/1
  In/1 -> To Workspace/1, Bus Selector2/1
  Bus Selector2/21 -> SteeringServo/1(In)  "<STEERC>"
  RightSpanServo/1(Out) -> Mux/16
  FlapRServo/1(Out) -> Mux/15
  LeftSpanServo/1(Out) -> Mux/14
  FlapLServo/1(Out) -> Mux/13
  RightOBSpoilerServo/1(Out) -> Mux/12
  RightIBSpoilerServo/1(Out) -> Mux/11
  LeftIBSpoilerServo/1(Out) -> Mux/9
  RudderLServo/1(Out) -> Mux/8
  Bus Selector2/12 -> RightOBSpoilerServo/1(In)  "<SPLROBC>"
  Bus Selector2/11 -> RightIBSpoilerServo/1(In)  "<SPLRIBC>"
  Bus Selector2/9 -> LeftIBSpoilerServo/1(In)  "<SPLLIBC>"
  Bus Selector2/8 -> RudderLServo/1(In)  "<RUDLOC>"
  Bus Selector2/7 -> RudderUServo/1(In)  "<RUDUPC>"
  RudderUServo/1(Out) -> Mux/7  "RUD"
  RightAileronServo/1(Out) -> Mux/6  "AILR"
  Bus Selector2/6 -> RightAileronServo/1(In)  "<AILRC>"
  LeftAileronServo/1(Out) -> Mux/5  "AILL"
  Bus Selector2/5 -> LeftAileronServo/1(In)  "<AILLC>"
  ElevatorRIBServo/1(Out) -> Mux/4
  Bus Selector2/4 -> ElevatorRIBServo/1(In)  "<ELRIBC>"
  ElevatorROBServo/1(Out) -> Mux/3
  Bus Selector2/3 -> ElevatorROBServo/1(In)  "<ELROBC>"
  ElevatorLIBServo/1(Out) -> Mux/2
  ElevatorLOBServo/1(Out) -> Mux/1  "ELL"
  Bus Selector2/2 -> ElevatorLIBServo/1(In)  "<ELLIBC>"
  Bus Selector2/1 -> ElevatorLOBServo/1(In)  "<ELLOBC>"
  Bus Selector2/18 -> Brake/1  "<BRAKEC>"
  Bus Selector2/16 -> RightSpanServo/1(In)  "<MORPHRC>"
  Bus Selector2/15 -> FlapRServo/1(In)  "<FLAPRC>"
  Bus Selector2/14 -> LeftSpanServo/1(In)  "<MORPHLC>"
  Bus Selector2/13 -> FlapLServo/1(In)  "<FLAPLC>"
  Bus Selector2/10 -> LeftOBSpoilerServo/1(In)  "<SPLLOBC>"
  LeftOBSpoilerServo/1(Out) -> Mux/10

== system gtm_design/GTM_T2/Actuators/DeadBand ==
  I : Inport
  Deadband : Subsystem
  Flaps : Constant  Value=SurfaceDeadbandOn
  Switch : Switch  Criteria=u2 ~= 0  Threshold=0.2
  O : Outport
  wires:
  I/1 -> Switch/3, Deadband/1(In)
  Deadband/1(Out) -> Switch/1
  Switch/1 -> O/1
  Flaps/1 -> Switch/2

== system gtm_design/GTM_T2/Actuators/InputModification for Trimming ==
  CmdVec : Inport
  SurfBias : Inport  Port=2
  SurfaceDeltas : Inport  Port=3
  Clock : Clock
  Compare To Constant : simulink/Logic and Bit Operations/Compare To Constant  relop=>=  const=0.2  OutDataTypeStr=boolean  ZeroCross=off
  Constant : Constant  Value=TrimModeOn
  Constant1 : Constant  Value=LinearizeModeOn
  Constant2 : Constant  Value=TrimModeOn
  Constant3 : Constant  Value=LinearizeModeOn
  Gain : Gain  Gain=2
  "Invalid, Error Out" : Subsystem  TreatAsAtomicUnit=on
  KillifNotSimMode : Assertion  AssertionFailFcn="warndlg('Running simulation with TrimMode or LinearizeMode engaged.  Run setup.m to reset.','Warning!')"
  LinearizeMode:DetlasOnTrimBias : Subsystem  TreatAsAtomicUnit=on
  Logical Operator : Logic  Operator=NAND  AllPortsSameDT=off  OutDataTypeStr=boolean
  Logical Operator1 : Logic  Operator=OR  AllPortsSameDT=off  OutDataTypeStr=boolean
  Merge : Merge  Inputs=4  InitialOutput=zeros(22,1)
  SimMode:PassThroughWithStab : Subsystem  TreatAsAtomicUnit=on
  Sum : Sum  Inputs=|++
  Switch Case : SwitchCase  CaseConditions={0,1,2}
  TrimMode: DriveFromTopLevel : Subsystem  TreatAsAtomicUnit=on
  CmdVecOut : Outport
  wires:
  "Invalid, Error Out"/1(Out) -> Merge/4
  Compare To Constant/1 -> Logical Operator/2
  Logical Operator1/1 -> Logical Operator/1
  Constant2/1 -> Logical Operator1/1
  Constant3/1 -> Logical Operator1/2
  Logical Operator/1 -> KillifNotSimMode/1
  Clock/1 -> Compare To Constant/1
  Switch Case/4 -> "Invalid, Error Out"/Action
  Sum/1 -> Switch Case/1
  Gain/1 -> Sum/2
  Constant/1 -> Sum/1
  Constant1/1 -> Gain/1
  LinearizeMode:DetlasOnTrimBias/1(Out) -> Merge/3
  SurfaceDeltas/1 -> LinearizeMode:DetlasOnTrimBias/1(In1)
  Switch Case/3 -> LinearizeMode:DetlasOnTrimBias/Action
  Merge/1 -> CmdVecOut/1
  TrimMode: DriveFromTopLevel/1(Out) -> Merge/2
  SimMode:PassThroughWithStab/1(Out) -> Merge/1
  SurfBias/1 -> TrimMode: DriveFromTopLevel/1(TrimBias)
  Switch Case/2 -> TrimMode: DriveFromTopLevel/Action
  Switch Case/1 -> SimMode:PassThroughWithStab/Action
  CmdVec/1 -> SimMode:PassThroughWithStab/1(Cmd)

== system gtm_design/GTM_T2/Actuators/Label ==
  I : Inport
  Bus Creator : BusCreator  Inputs=22
  Demux : Demux  Outputs=22
  O : Outport
  wires:
  Demux/22 -> Bus Creator/22  "STEER"
  Demux/21 -> Bus Creator/21  "THROTR"
  Demux/20 -> Bus Creator/20  "THROTL"
  Demux/19 -> Bus Creator/19  "BRAKE"
  Demux/1 -> Bus Creator/1  "ELLOB"
  Demux/18 -> Bus Creator/18  "GEAR"
  Demux/17 -> Bus Creator/17  "STAB"
  Demux/16 -> Bus Creator/16  "FLAPROB"
  Demux/15 -> Bus Creator/15  "FLAPRIB"
  Demux/14 -> Bus Creator/14  "FLAPLOB"
  Demux/13 -> Bus Creator/13  "FLAPLIB"
  Demux/12 -> Bus Creator/12  "SPLROB"
  Demux/11 -> Bus Creator/11  "SPLRIB"
  Demux/10 -> Bus Creator/10  "SPLLOB"
  Demux/9 -> Bus Creator/9  "SPLLIB"
  Demux/8 -> Bus Creator/8  "RUDL"
  Demux/7 -> Bus Creator/7  "RUDU"
  Demux/6 -> Bus Creator/6  "AILR"
  Demux/5 -> Bus Creator/5  "AILL"
  Demux/4 -> Bus Creator/4  "ELRIB"
  Demux/3 -> Bus Creator/3  "ELROB"
  Demux/2 -> Bus Creator/2  "ELLIB"
  Bus Creator/1 -> O/1
  I/1 -> Demux/1

== system gtm_design/GTM_T2/Actuators/TimeDelay with IC feedthrough ==
  I : Inport
  Clock : Clock
  Demux : Demux  Outputs=[16 5]
  Mux : Mux  Inputs=[16 5]
  Switch : Switch  Threshold=10.1e-3
  Transport Delay : TransportDelay  DelayTime=10e-3
      settings: AttributesFormatString=%<DelayTime>
  O : Outport
  wires:
  Mux/1 -> Switch/1
  Demux/2 -> Mux/2
  Transport Delay/1 -> Mux/1
  Demux/1 -> Transport Delay/1
  Switch/1 -> O/1
  Clock/1 -> Switch/2
  I/1 -> Demux/1, Switch/3

== system gtm_design/GTM_T2/Aero/Basic Airframe ==
  note: The basic aerodynamics are asymmetric.
      | When the 'symmetry_on' flag is set, increments
      | from the dC3_sym aero table are added to the
      | lateral-directional coefficients (CY,Cl,Cn) to make
      | them symmetric.  When the flag is off, the gain of
      | 2.0 is applied to the increments,which effectively
      | changes the sign of the asymmetries.
  alpha : Inport
  beta : Inport  Port=2
  symmetry_on : Inport  Port=3
  AC_Params : Inport  Port=4
  Add : Sum  Inputs=+++
  AlphaLookup : PreLookup  BreakpointsData=Aero.C6_bas.alpha  IndexSearchMethod=Linear search  BeginIndexSearchUsingPreviousIndexResult=on  ExtrapMethod=Linear
  AlphaLookup1 : PreLookup  BreakpointsData=Aero.C6_bas.beta  IndexSearchMethod=Linear search  BeginIndexSearchUsingPreviousIndexResult=on  ExtrapMethod=Linear
  Assignment to Lateral : Assignment  IndexMode=Zero-based  IndexOptions=Index vector (dialog)  Indices=[1 3 5]  OutputSizes=[1 1]
  Bus Selector : BusSelector  OutputSignals=DamageCase
  Constant : Constant  Value=zeros(6,1)
  Constant1 : Constant  Value=[0:5]  OutDataTypeStr=uint32
  Constant2 : Constant  Value=[0:2]  OutDataTypeStr=uint32
  DamageEffects : Subsystem
  Data Type Conversion : DataTypeConversion  OutDataTypeStr=uint32  RndMeth=Nearest
  Gain : Gain  Gain=2
  Interpolation Using Prelookup : Interpolation_n-D  NumberOfTableDimensions=3  Table=Aero.C6_bas.data  NumSelectionDims=1
      settings: InputPortMap=u0,u1,u2,u3,u4
  Interpolation Using Prelookup1 : Interpolation_n-D  NumberOfTableDimensions=3  Table=Aero.dC3_sym.data  NumSelectionDims=1
      settings: InputPortMap=u0,u1,u2,u3,u4
  Switch : Switch  Criteria=u2 ~= 0
  C6 : Outport
  wires:
  Assignment to Lateral/1 -> Gain/1, Switch/1
  Data Type Conversion/1 -> DamageEffects/3(damage_case)
  Constant2/1 -> Interpolation Using Prelookup1/5
  Constant1/1 -> Interpolation Using Prelookup/5
  AlphaLookup1/2 -> Interpolation Using Prelookup1/4, Interpolation Using Prelookup/4
  AlphaLookup1/1 -> Interpolation Using Prelookup1/3, Interpolation Using Prelookup/3
  AlphaLookup/2 -> Interpolation Using Prelookup1/2, Interpolation Using Prelookup/2
  AlphaLookup/1 -> Interpolation Using Prelookup1/1, Interpolation Using Prelookup/1
  Bus Selector/1 -> Data Type Conversion/1  "<DamageCase>"
  AC_Params/1 -> Bus Selector/1
  DamageEffects/1(dC6_dam) -> Add/3
  beta/1 -> AlphaLookup1/1, DamageEffects/2(beta)
  alpha/1 -> AlphaLookup/1, DamageEffects/1(alpha)
  Switch/1 -> Add/2
  Add/1 -> C6/1
  symmetry_on/1 -> Switch/2
  Gain/1 -> Switch/3
  Interpolation Using Prelookup1/1 -> Assignment to Lateral/2
  Constant/1 -> Assignment to Lateral/1
  Interpolation Using Prelookup/1 -> Add/1

== system gtm_design/GTM_T2/Aero/Coefficent Evaluation ==
  C6 Body : Inport
  qbar : Inport  Port=2
  Cg : Inport  Port=3
  Cp : Inport  Port=4
  3D Vector Cross Product : Subsystem
  Demux : Demux  Outputs=[3 3]
      settings: DisplayOption=none
  Gain2 : Gain  Gain=Sref  SaturateOnIntegerOverflow=on  OutDataTypeStr=Inherit: Same as input  ParamDataTypeStr=Inherit: Same as input
  Product : Product  InputSameDT=on  SaturateOnIntegerOverflow=on  OutDataTypeStr=Inherit: Same as first input
  Reference Lengths : Gain  Gain=[b cbar b]  SaturateOnIntegerOverflow=on  OutDataTypeStr=Inherit: Same as input  ParamDataTypeStr=Inherit: Same as input
  Sum : Sum  Inputs=-+  SaturateOnIntegerOverflow=on
  Sum1 : Sum  Inputs=++|  SaturateOnIntegerOverflow=on
  Forces : Outport
  Moments : Outport  Port=2
  wires:
  3D Vector Cross Product/1(AxB) -> Sum1/1
  Sum1/1 -> Moments/1
  Reference Lengths/1 -> Sum1/2
  Demux/1 -> Forces/1, 3D Vector Cross Product/2(B)
  Demux/2 -> Reference Lengths/1
  Gain2/1 -> Demux/1
  Product/1 -> Gain2/1
  qbar/1 -> Product/2
  C6 Body/1 -> Product/1
  Cp/1 -> Sum/2
  Cg/1 -> Sum/1
  Sum/1 -> 3D Vector Cross Product/1(A)
